simulink model "CLosed_loop_buck_PID2"  (Simulink 7.7)
settings: Solver=FixedStepDiscrete  SolverMode=SingleTasking  StartTime=0.0  StopTime=0.2  FixedStep=0.0000001  RelTol=1e-3
undefined symbols (not defined in the file or in its folder): OC2max
libraries: dsPICdrivers x7, simulink x1
settings Model: Creator=Lubin  LastModifiedBy=More
settings OptimizationCC: InitFltsAndDblsToZero=on  OptimizeModelRefInitCode=on  LifeSpan=1
settings DebuggingCC: SaveWithParameterizedLinksMsg=none  SignalResolutionControl=TryResolveAllWithWarning  StrictBusMsg=Warning
settings HardwareCC: ProdBitPerInt=16  ProdBitPerPointer=16  ProdEndianess=LittleEndian  ProdWordSize=16  ProdHWDeviceType=16-bit Generic  TargetHWDeviceType=32-bit Generic
settings RTWCC: SystemTargetFile=dspic.tlc  MakeCommand=make_CreateMPLAB  TemplateMakefile=dspic_pic30_gcc.tmf  PostCodeGenCommand=dsPIC_Compile()  Description=Embedded Target for Microchip dsPIC (real-time)  ProcessScript=dspic_make_rtw_hook
settings CodeAppCC: IgnoreCustomStorageClasses=off
settings STFCustomTargetCC: TargetFcnLib=ansi_tfl_tmw.mat  FunctionExecutionProfile=off  IncludeMdlTerminateFcn=off  CombineOutputUpdateFcns=on  SuppressErrorStatus=on  ERTCustomFileBanners=on  SupportNonFinite=off  SupportComplex=off  SupportContinuousTime=off  SupportNonInlinedSFcns=off  CPPClassGenCompliant=on  SystemTargetFile=dspic.tlc
settings ERTTargetCC: TargetFcnLib=ansi_tfl_tmw.mat  FunctionExecutionProfile=off  MultiwordLength=2048  ParMdlRefBuildCompliant=off  CompOptLevelCompliant=off  IncludeMdlTerminateFcn=off  SuppressErrorStatus=on  ERTFirstTimeCompliant=off  SupportNonFinite=off  SupportComplex=off  ModelStepFunctionPrototypeControlCompliant=off  ExtModeMexFile=ext_serial_win32_comm  InlinedParameterPlacement=NonHierarchical  ERTSrcFileBannerTemplate=dsPIC_code_template.cgt  ERTHdrFileBannerTemplate=dsPIC_code_template.cgt  ERTDataSrcFileTemplate=dsPIC_code_template.cgt  ERTDataHdrFileTemplate=dsPIC_code_template.cgt  ERTCustomFileTemplate=dsPIC_main.tlc  ConvertIfToSwitch=off
settings CustomProperty: DataType=string  Value=C:\PROGRA~1\MATLAB\R2011a\bin\win64\gmake

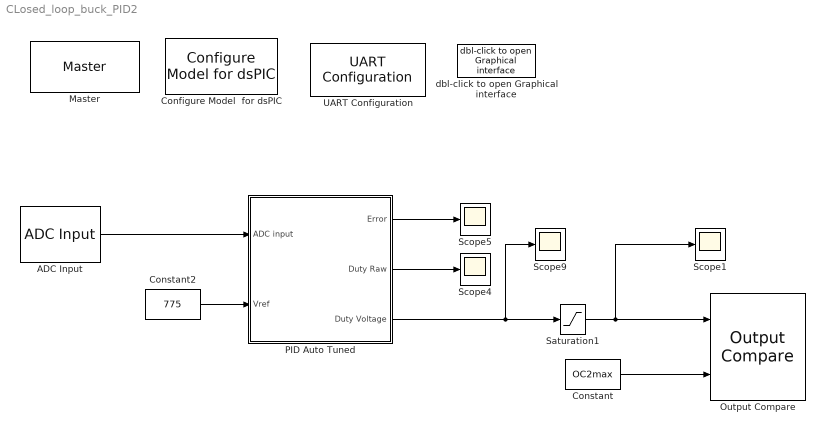
== system CLosed_loop_buck_PID2 ==
  ADC Input : dsPICdrivers/Peripheral I//O/ADC Input  Tag=dsPIC_ADC  Priority=5  ADC_TYPE=10 bits  ADC_MODE=Continuous sampling & get last channel value  NbrSampleStep=1  VoltRefpopup="AVdd  -  AVss"  OutFormatBitspopup=0000 00dd dddd dddd : Integer  InterruptPriority=6  ANCHANNELS=[3]  MaxName=ANmax = 1023  Rin=1e2  ADCS=4  SAMC=1  Temperature=25  DMAChannel=7  SampleTime=1/10000  Status="OK  |  Tsmp=1.563e-007 |  T/Channel=2.031e-006 |  Tall=2.031e-006"  SSRC=Low to High transition on INT0 pin
  Configure Model  for dsPIC : dsPICdrivers/Simulink Configuration/Configure Model  for dsPIC
  Constant : Constant  Value=OC2max  OutDataTypeStr=uint16
  Constant2 : Constant  Value=775  OutDataTypeStr=uint16  SampleTime=1/10000
  Master : dsPICdrivers/Master  Tag=dsPIC_MASTER  Priority=1  TimeStepType=Timer1  picType=24fJ128GA010  fcy=16000000  Quartz_33f=8e6  PLLActive_33f=on  fcyDesired_33f=0  tmr1="[1  1  -25]"  tmr1Info="Time Step : 1.25e-007  ;   Error : -25%  PR1=1"  tmr2345="[1  0  0  0]"  tmr2345cfg=[-1 -1 -1 -1]  IOautoConf=on  typePort="[ 0  0  0  0  0  0  0  0  0  0  0  0  0  0  0  0  0  0  0  8  0  0  0  0  0  0  0  0  0  0  0  0  0  0  0  0  0  0  0  0  0  0  0  0  0  0  0  0  0  7  0  0  0  0  0  0  0  0  0  0  0  0  0  0  0  0  0  0  0  0  0  0  0  0  0  0  0  0  0  0  0  0  0  0  4  5  0  0  0  0  0  0  0  0  0  0  0  0  0  0  0  0  0  0  0  0  0  0  0  0  0  0 ]"  TRIS="[ 65535  65535  65535  65533  65535  65535  65535 ]"  ADPCFG=0  MasterBusyPort=None  MasterOverloadPort=None  FOSC=Quartz (XT - HS)  ClockSwitchMonitor=Both disabled  TempProtection_33f=TEMP_ON  FPBOR=<empty>  PWRT=disable  MCLR=<empty>  ICD=ICS_PGD1  JTAGEN=JTAGEN_OFF  PowerSave=off  OverrideFcy=off  NewFcy=1e6  PR2345="[65535  65535  65535  65535]"
  Output Compare : dsPICdrivers/Peripheral I//O/Output Compare  Tag=dsPIC_PWM_out  Priority=5  IntPriority=1  CHANNEL=[2]  Channel_UP_Down_Periode=[5]  MaxChannel=[2e-005]  MaxName=' OC2max '  Precision=[8.3129]  Timer=[2]  Status=OK  SafeMarge=[0]  PortLetter=[68]  PortNumber=[1]  MaxValues=[319]
  PID Auto Tuned : Subsystem
  Saturation1 : Saturate  UpperLimit=160  LowerLimit=10  LinearizeAsGain=off  OutDataTypeStr=uint16
  Scope{1,4..5,9} (4 alike) : Scope
      Scope1 settings: YMin=72.5  YMax=112.5
      Scope4 settings: TimeRange=0.018  SaveName=ScopeData2
      Scope5 settings: TimeRange=0.018  SaveName=ScopeData3
      Scope9 settings: TimeRange=0.018  SaveName=ScopeData9
  UART Configuration : dsPICdrivers/Serial PORT/UART Configuration  Tag=dsPIC_config_UART  Priority=2  UART=2  proposed_BAUD=19200  BAUD=19200  ALT_TX_RX=off  InterruptTxWhen=When Transmit Buffer is empty  TXInterruptPri=7  TxBufferSize=32  TXEN=on  InterruptRxWhen=When Receive Buffer is full (contain 4 characters)  RXInterruptPri=1  RxBufferSize=32  DoNotImplementRxInterrupt=off  DoNotImplementTxInterrupt=off  UxBRG=51  Info="UxBRG = 51   ||  Real Baud : 19231   ||  % error : 0.16026  ||  max 0.00019231 Bytes / Step"  RealBaud=0  ERROR=0.16026  BYTES_STEP=0.00019231
  dbl-click to open Graphical interface : dsPICdrivers/Serial PORT/dbl-click to open Graphical interface  Nothing=0
  wires:
  Constant2/1 -> PID Auto Tuned/2(Vref)
  Constant/1 -> Output Compare/2
  Saturation1/1 -> Scope1/1, Output Compare/1
  PID Auto Tuned/3(Duty Voltage) -> Saturation1/1, Scope9/1
  PID Auto Tuned/1(Error) -> Scope5/1
  PID Auto Tuned/2(Duty Raw) -> Scope4/1
  ADC Input/1 -> PID Auto Tuned/1(ADC input)

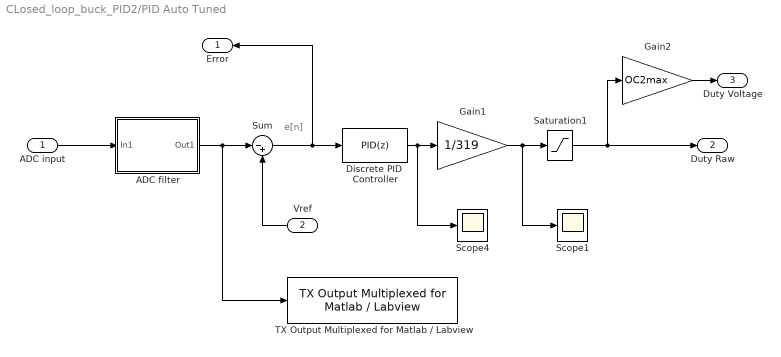
== system CLosed_loop_buck_PID2/PID Auto Tuned ==
  note: e[n]
  ADC input : Inport
  Vref : Inport  Port=2
  ADC filter : Subsystem
  Discrete PID  Controller : simulink/Continuous/PID Controller  SystemSampleTime=-1  Controller=PID  TimeDomain=Discrete-time  SampleTime=1/10000  IntegratorMethod=Forward Euler  FilterMethod=Forward Euler  Form=Parallel  P=0.634971329771802  I=160.765194841517  D=0.000367278724120311  N=13291.0514556826  InitialConditionSource=internal  InitialConditionForIntegrator=0  InitialConditionForFilter=0  ExternalReset=none  LimitOutput=off  UpperSaturationLimit=319  LowerSaturationLimit=0  LinearizeAsGain=off  AntiWindupMode=none  Kb=1  TrackingMode=off  Kt=1  SaturateOnIntegerOverflow=on  PParamMin=[]  PParamMax=[]  PParamDataTypeStr=double  IParamMin=[]  IParamMax=[]  IParamDataTypeStr=double  DParamMin=[]  DParamMax=[]  DParamDataTypeStr=double  NParamMin=[]  NParamMax=[]  NParamDataTypeStr=double  KbParamMin=[]  KbParamMax=[]  KtParamMin=[]  KtParamMax=[]  POutMin=[]  POutMax=[]  POutDataTypeStr=double  IOutMin=[]  IOutMax=[]  IOutDataTypeStr=double  DOutMin=[]  DOutMax=[]  DOutDataTypeStr=double  NOutMin=[]  NOutMax=[]  NOutDataTypeStr=double  KbOutMin=[]  KbOutMax=[]  KtOutMin=[]  KtOutMax=[]  IntegratorOutMin=[]  IntegratorOutMax=[]  IntegratorOutDataTypeStr=double  FilterOutMin=[]  FilterOutMax=[]  FilterOutDataTypeStr=double  SumOutMin=[]  SumOutMax=[]  SumOutDataTypeStr=double  SumI1OutMin=[]  SumI1OutMax=[]  SumI2OutMin=[]  SumI2OutMax=[]  SumI3OutMin=[]  SumI3OutMax=[]  SumDOutMin=[]  SumDOutMax=[]  SumDOutDataTypeStr=double  SumAccumDataTypeStr=double  SumDAccumDataTypeStr=double  SaturationOutMin=[]  SaturationOutMax=[]  IntegratorContinuousStateAttributes=''  IntegratorStateMustResolveToSignalObject=off  IntegratorRTWStateStorageClass=Auto  FilterContinuousStateAttributes=''  FilterStateMustResolveToSignalObject=off  FilterRTWStateStorageClass=Auto
      settings: LockScale=on
  Gain1 : Gain  Gain=1/319  OutDataTypeStr=double  SampleTime=1/10000
  Gain2 : Gain  Gain=OC2max  OutDataTypeStr=double  SampleTime=1/10000
  Saturation1 : Saturate  UpperLimit=0.99  LowerLimit=0  LinearizeAsGain=off  SampleTime=1/10000  OutDataTypeStr=double
  Scope1 : Scope
      settings: TimeRange=0.018  SaveName=ScopeData4
  Scope4 : Scope
      settings: TimeRange=0.018
  Sum : Sum  Inputs=|-+  OutDataTypeStr=int16  SampleTime=1/20000
  TX Output Multiplexed for Matlab / Labview : dsPICdrivers/Serial PORT/TX Output Multiplexed for Matlab // Labview  Tag=dsPIC_TX_Multiplexed  Priority=5  UART=2  CleverSpreadingChk=on  CleverSpreading=1  CHANNEL=[0]  CHANNELBLOCKED=[]  CHANNELBLOCKED_BITEWISE=0  Status=OK
  Error : Outport
  Duty Raw : Outport  Port=2
  Duty Voltage : Outport  Port=3
  wires:
  Gain2/1 -> Duty Voltage/1
  ADC input/1 -> ADC filter/1(In1)
  Vref/1 -> Sum/2
  Sum/1 -> Error/1, Discrete PID  Controller/1
  Discrete PID  Controller/1 -> Gain1/1, Scope4/1
  Saturation1/1 -> Duty Raw/1, Gain2/1
  Gain1/1 -> Saturation1/1, Scope1/1
  ADC filter/1(Out1) -> Sum/1, TX Output Multiplexed for Matlab / Labview/1

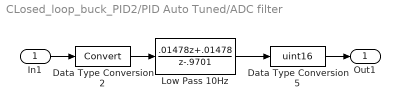
== system CLosed_loop_buck_PID2/PID Auto Tuned/ADC filter ==
  In1 : Inport
  Data Type Conversion2 : DataTypeConversion
  Data Type Conversion5 : DataTypeConversion  OutDataTypeStr=uint16
  Low Pass 10Hz : DiscreteTransferFcn  Numerator=[.01478 .01478]  Denominator=[1 -.9701]  SampleTime=-1
  Out1 : Outport
  wires:
  Data Type Conversion2/1 -> Low Pass 10Hz/1
  Low Pass 10Hz/1 -> Data Type Conversion5/1
  In1/1 -> Data Type Conversion2/1
  Data Type Conversion5/1 -> Out1/1
